simulink model "rfsoc4x2_ospfb_128"  (R2021a)
settings: Solver=VariableStepAuto  StartTime=0.0  StopTime=2048  RelTol=1e-3
undefined symbols (not defined in the file): pfb_coeff_gen_calc
libraries: xbsIndex_r4 x37092, casper_library_delays x737, casper_library_misc x68, xps_library x1
(part 232 of 339)

== system rfsoc4x2_ospfb_128/fft_wideband_real1/fft_direct/butterfly1_1/bus_convert/conv11 ==
  din : Inport
  all_0s : xbsIndex_r4/Logical  logical_function=NAND  inputs=3  en=off  latency=2  precision=Full  arith_type=Unsigned  n_bits=16  bin_pt=0  align_bp=on  dbl_ovrd=off  block_type=logical
  all_1s : xbsIndex_r4/Logical  logical_function=NAND  inputs=3  en=off  latency=2  precision=Full  arith_type=Unsigned  n_bits=16  bin_pt=0  align_bp=on  dbl_ovrd=off  block_type=logical
  and : xbsIndex_r4/Logical  logical_function=AND  inputs=2  en=off  latency=1  precision=Full  arith_type=Unsigned  n_bits=16  bin_pt=0  align_bp=on  dbl_ovrd=off  block_type=logical
  convert : xbsIndex_r4/Convert  gui_display_data_type=Fixed-point  arith_type="Signed  (2's comp)"  n_bits=bit_width_o  bin_pt=binary_point_o  float_type=Single  exp_bits=8  fraction_bits=24  quantization="Round  (unbiased: +/- Inf)"  overflow=Wrap  en=off  latency=csp_latency  pipeline=on  dbl_ovrd=off  block_type=convert
  invert1 : xbsIndex_r4/Inverter  en=off  latency=0  dbl_ovrd=off  block_type=inv
  invert2 : xbsIndex_r4/Inverter  en=off  latency=0  dbl_ovrd=off  block_type=inv
  invert3 : xbsIndex_r4/Inverter  en=off  latency=0  dbl_ovrd=off  block_type=inv
  slice1 : xbsIndex_r4/Slice  nbits=1  boolean_output=on  mode=Upper Bit Location + Width  bit1=0  base1=MSB of Input  bit0=0  base0=LSB of Input  dbl_ovrd=off  block_type=slice
  slice2 : xbsIndex_r4/Slice  nbits=1  boolean_output=on  mode=Upper Bit Location + Width  bit1=-1  base1=MSB of Input  bit0=0  base0=LSB of Input  dbl_ovrd=off  block_type=slice
  slice3 : xbsIndex_r4/Slice  nbits=1  boolean_output=on  mode=Upper Bit Location + Width  bit1=-2  base1=MSB of Input  bit0=0  base0=LSB of Input  dbl_ovrd=off  block_type=slice
  dout : Outport
  of : Outport  Port=2
  wires:
  and/1 -> of/1
  all_1s/1 -> and/2
  all_0s/1 -> and/1
  invert3/1 -> all_0s/3
  slice3/1 -> invert3/1, all_1s/3
  invert2/1 -> all_0s/2
  slice2/1 -> invert2/1, all_1s/2
  invert1/1 -> all_0s/1
  slice1/1 -> invert1/1, all_1s/1
  convert/1 -> dout/1
  din/1 -> slice3/1, slice2/1, slice1/1, convert/1

== system rfsoc4x2_ospfb_128/fft_wideband_real1/fft_direct/butterfly1_1/bus_convert/conv12 ==
  din : Inport
  all_0s : xbsIndex_r4/Logical  logical_function=NAND  inputs=3  en=off  latency=2  precision=Full  arith_type=Unsigned  n_bits=16  bin_pt=0  align_bp=on  dbl_ovrd=off  block_type=logical
  all_1s : xbsIndex_r4/Logical  logical_function=NAND  inputs=3  en=off  latency=2  precision=Full  arith_type=Unsigned  n_bits=16  bin_pt=0  align_bp=on  dbl_ovrd=off  block_type=logical
  and : xbsIndex_r4/Logical  logical_function=AND  inputs=2  en=off  latency=1  precision=Full  arith_type=Unsigned  n_bits=16  bin_pt=0  align_bp=on  dbl_ovrd=off  block_type=logical
  convert : xbsIndex_r4/Convert  gui_display_data_type=Fixed-point  arith_type="Signed  (2's comp)"  n_bits=bit_width_o  bin_pt=binary_point_o  float_type=Single  exp_bits=8  fraction_bits=24  quantization="Round  (unbiased: +/- Inf)"  overflow=Wrap  en=off  latency=csp_latency  pipeline=on  dbl_ovrd=off  block_type=convert
  invert1 : xbsIndex_r4/Inverter  en=off  latency=0  dbl_ovrd=off  block_type=inv
  invert2 : xbsIndex_r4/Inverter  en=off  latency=0  dbl_ovrd=off  block_type=inv
  invert3 : xbsIndex_r4/Inverter  en=off  latency=0  dbl_ovrd=off  block_type=inv
  slice1 : xbsIndex_r4/Slice  nbits=1  boolean_output=on  mode=Upper Bit Location + Width  bit1=0  base1=MSB of Input  bit0=0  base0=LSB of Input  dbl_ovrd=off  block_type=slice
  slice2 : xbsIndex_r4/Slice  nbits=1  boolean_output=on  mode=Upper Bit Location + Width  bit1=-1  base1=MSB of Input  bit0=0  base0=LSB of Input  dbl_ovrd=off  block_type=slice
  slice3 : xbsIndex_r4/Slice  nbits=1  boolean_output=on  mode=Upper Bit Location + Width  bit1=-2  base1=MSB of Input  bit0=0  base0=LSB of Input  dbl_ovrd=off  block_type=slice
  dout : Outport
  of : Outport  Port=2
  wires:
  and/1 -> of/1
  all_1s/1 -> and/2
  all_0s/1 -> and/1
  invert3/1 -> all_0s/3
  slice3/1 -> invert3/1, all_1s/3
  invert2/1 -> all_0s/2
  slice2/1 -> invert2/1, all_1s/2
  invert1/1 -> all_0s/1
  slice1/1 -> invert1/1, all_1s/1
  convert/1 -> dout/1
  din/1 -> slice3/1, slice2/1, slice1/1, convert/1

== system rfsoc4x2_ospfb_128/fft_wideband_real1/fft_direct/butterfly1_1/bus_convert/conv13 ==
  din : Inport
  all_0s : xbsIndex_r4/Logical  logical_function=NAND  inputs=3  en=off  latency=2  precision=Full  arith_type=Unsigned  n_bits=16  bin_pt=0  align_bp=on  dbl_ovrd=off  block_type=logical
  all_1s : xbsIndex_r4/Logical  logical_function=NAND  inputs=3  en=off  latency=2  precision=Full  arith_type=Unsigned  n_bits=16  bin_pt=0  align_bp=on  dbl_ovrd=off  block_type=logical
  and : xbsIndex_r4/Logical  logical_function=AND  inputs=2  en=off  latency=1  precision=Full  arith_type=Unsigned  n_bits=16  bin_pt=0  align_bp=on  dbl_ovrd=off  block_type=logical
  convert : xbsIndex_r4/Convert  gui_display_data_type=Fixed-point  arith_type="Signed  (2's comp)"  n_bits=bit_width_o  bin_pt=binary_point_o  float_type=Single  exp_bits=8  fraction_bits=24  quantization="Round  (unbiased: +/- Inf)"  overflow=Wrap  en=off  latency=csp_latency  pipeline=on  dbl_ovrd=off  block_type=convert
  invert1 : xbsIndex_r4/Inverter  en=off  latency=0  dbl_ovrd=off  block_type=inv
  invert2 : xbsIndex_r4/Inverter  en=off  latency=0  dbl_ovrd=off  block_type=inv
  invert3 : xbsIndex_r4/Inverter  en=off  latency=0  dbl_ovrd=off  block_type=inv
  slice1 : xbsIndex_r4/Slice  nbits=1  boolean_output=on  mode=Upper Bit Location + Width  bit1=0  base1=MSB of Input  bit0=0  base0=LSB of Input  dbl_ovrd=off  block_type=slice
  slice2 : xbsIndex_r4/Slice  nbits=1  boolean_output=on  mode=Upper Bit Location + Width  bit1=-1  base1=MSB of Input  bit0=0  base0=LSB of Input  dbl_ovrd=off  block_type=slice
  slice3 : xbsIndex_r4/Slice  nbits=1  boolean_output=on  mode=Upper Bit Location + Width  bit1=-2  base1=MSB of Input  bit0=0  base0=LSB of Input  dbl_ovrd=off  block_type=slice
  dout : Outport
  of : Outport  Port=2
  wires:
  and/1 -> of/1
  all_1s/1 -> and/2
  all_0s/1 -> and/1
  invert3/1 -> all_0s/3
  slice3/1 -> invert3/1, all_1s/3
  invert2/1 -> all_0s/2
  slice2/1 -> invert2/1, all_1s/2
  invert1/1 -> all_0s/1
  slice1/1 -> invert1/1, all_1s/1
  convert/1 -> dout/1
  din/1 -> slice3/1, slice2/1, slice1/1, convert/1

== system rfsoc4x2_ospfb_128/fft_wideband_real1/fft_direct/butterfly1_1/bus_convert/conv14 ==
  din : Inport
  all_0s : xbsIndex_r4/Logical  logical_function=NAND  inputs=3  en=off  latency=2  precision=Full  arith_type=Unsigned  n_bits=16  bin_pt=0  align_bp=on  dbl_ovrd=off  block_type=logical
  all_1s : xbsIndex_r4/Logical  logical_function=NAND  inputs=3  en=off  latency=2  precision=Full  arith_type=Unsigned  n_bits=16  bin_pt=0  align_bp=on  dbl_ovrd=off  block_type=logical
  and : xbsIndex_r4/Logical  logical_function=AND  inputs=2  en=off  latency=1  precision=Full  arith_type=Unsigned  n_bits=16  bin_pt=0  align_bp=on  dbl_ovrd=off  block_type=logical
  convert : xbsIndex_r4/Convert  gui_display_data_type=Fixed-point  arith_type="Signed  (2's comp)"  n_bits=bit_width_o  bin_pt=binary_point_o  float_type=Single  exp_bits=8  fraction_bits=24  quantization="Round  (unbiased: +/- Inf)"  overflow=Wrap  en=off  latency=csp_latency  pipeline=on  dbl_ovrd=off  block_type=convert
  invert1 : xbsIndex_r4/Inverter  en=off  latency=0  dbl_ovrd=off  block_type=inv
  invert2 : xbsIndex_r4/Inverter  en=off  latency=0  dbl_ovrd=off  block_type=inv
  invert3 : xbsIndex_r4/Inverter  en=off  latency=0  dbl_ovrd=off  block_type=inv
  slice1 : xbsIndex_r4/Slice  nbits=1  boolean_output=on  mode=Upper Bit Location + Width  bit1=0  base1=MSB of Input  bit0=0  base0=LSB of Input  dbl_ovrd=off  block_type=slice
  slice2 : xbsIndex_r4/Slice  nbits=1  boolean_output=on  mode=Upper Bit Location + Width  bit1=-1  base1=MSB of Input  bit0=0  base0=LSB of Input  dbl_ovrd=off  block_type=slice
  slice3 : xbsIndex_r4/Slice  nbits=1  boolean_output=on  mode=Upper Bit Location + Width  bit1=-2  base1=MSB of Input  bit0=0  base0=LSB of Input  dbl_ovrd=off  block_type=slice
  dout : Outport
  of : Outport  Port=2
  wires:
  and/1 -> of/1
  all_1s/1 -> and/2
  all_0s/1 -> and/1
  invert3/1 -> all_0s/3
  slice3/1 -> invert3/1, all_1s/3
  invert2/1 -> all_0s/2
  slice2/1 -> invert2/1, all_1s/2
  invert1/1 -> all_0s/1
  slice1/1 -> invert1/1, all_1s/1
  convert/1 -> dout/1
  din/1 -> slice3/1, slice2/1, slice1/1, convert/1

== system rfsoc4x2_ospfb_128/fft_wideband_real1/fft_direct/butterfly1_1/bus_convert/conv15 ==
  din : Inport
  all_0s : xbsIndex_r4/Logical  logical_function=NAND  inputs=3  en=off  latency=2  precision=Full  arith_type=Unsigned  n_bits=16  bin_pt=0  align_bp=on  dbl_ovrd=off  block_type=logical
  all_1s : xbsIndex_r4/Logical  logical_function=NAND  inputs=3  en=off  latency=2  precision=Full  arith_type=Unsigned  n_bits=16  bin_pt=0  align_bp=on  dbl_ovrd=off  block_type=logical
  and : xbsIndex_r4/Logical  logical_function=AND  inputs=2  en=off  latency=1  precision=Full  arith_type=Unsigned  n_bits=16  bin_pt=0  align_bp=on  dbl_ovrd=off  block_type=logical
  convert : xbsIndex_r4/Convert  gui_display_data_type=Fixed-point  arith_type="Signed  (2's comp)"  n_bits=bit_width_o  bin_pt=binary_point_o  float_type=Single  exp_bits=8  fraction_bits=24  quantization="Round  (unbiased: +/- Inf)"  overflow=Wrap  en=off  latency=csp_latency  pipeline=on  dbl_ovrd=off  block_type=convert
  invert1 : xbsIndex_r4/Inverter  en=off  latency=0  dbl_ovrd=off  block_type=inv
  invert2 : xbsIndex_r4/Inverter  en=off  latency=0  dbl_ovrd=off  block_type=inv
  invert3 : xbsIndex_r4/Inverter  en=off  latency=0  dbl_ovrd=off  block_type=inv
  slice1 : xbsIndex_r4/Slice  nbits=1  boolean_output=on  mode=Upper Bit Location + Width  bit1=0  base1=MSB of Input  bit0=0  base0=LSB of Input  dbl_ovrd=off  block_type=slice
  slice2 : xbsIndex_r4/Slice  nbits=1  boolean_output=on  mode=Upper Bit Location + Width  bit1=-1  base1=MSB of Input  bit0=0  base0=LSB of Input  dbl_ovrd=off  block_type=slice
  slice3 : xbsIndex_r4/Slice  nbits=1  boolean_output=on  mode=Upper Bit Location + Width  bit1=-2  base1=MSB of Input  bit0=0  base0=LSB of Input  dbl_ovrd=off  block_type=slice
  dout : Outport
  of : Outport  Port=2
  wires:
  and/1 -> of/1
  all_1s/1 -> and/2
  all_0s/1 -> and/1
  invert3/1 -> all_0s/3
  slice3/1 -> invert3/1, all_1s/3
  invert2/1 -> all_0s/2
  slice2/1 -> invert2/1, all_1s/2
  invert1/1 -> all_0s/1
  slice1/1 -> invert1/1, all_1s/1
  convert/1 -> dout/1
  din/1 -> slice3/1, slice2/1, slice1/1, convert/1

== system rfsoc4x2_ospfb_128/fft_wideband_real1/fft_direct/butterfly1_1/bus_convert/conv16 ==
  din : Inport
  all_0s : xbsIndex_r4/Logical  logical_function=NAND  inputs=3  en=off  latency=2  precision=Full  arith_type=Unsigned  n_bits=16  bin_pt=0  align_bp=on  dbl_ovrd=off  block_type=logical
  all_1s : xbsIndex_r4/Logical  logical_function=NAND  inputs=3  en=off  latency=2  precision=Full  arith_type=Unsigned  n_bits=16  bin_pt=0  align_bp=on  dbl_ovrd=off  block_type=logical
  and : xbsIndex_r4/Logical  logical_function=AND  inputs=2  en=off  latency=1  precision=Full  arith_type=Unsigned  n_bits=16  bin_pt=0  align_bp=on  dbl_ovrd=off  block_type=logical
  convert : xbsIndex_r4/Convert  gui_display_data_type=Fixed-point  arith_type="Signed  (2's comp)"  n_bits=bit_width_o  bin_pt=binary_point_o  float_type=Single  exp_bits=8  fraction_bits=24  quantization="Round  (unbiased: +/- Inf)"  overflow=Wrap  en=off  latency=csp_latency  pipeline=on  dbl_ovrd=off  block_type=convert
  invert1 : xbsIndex_r4/Inverter  en=off  latency=0  dbl_ovrd=off  block_type=inv
  invert2 : xbsIndex_r4/Inverter  en=off  latency=0  dbl_ovrd=off  block_type=inv
  invert3 : xbsIndex_r4/Inverter  en=off  latency=0  dbl_ovrd=off  block_type=inv
  slice1 : xbsIndex_r4/Slice  nbits=1  boolean_output=on  mode=Upper Bit Location + Width  bit1=0  base1=MSB of Input  bit0=0  base0=LSB of Input  dbl_ovrd=off  block_type=slice
  slice2 : xbsIndex_r4/Slice  nbits=1  boolean_output=on  mode=Upper Bit Location + Width  bit1=-1  base1=MSB of Input  bit0=0  base0=LSB of Input  dbl_ovrd=off  block_type=slice
  slice3 : xbsIndex_r4/Slice  nbits=1  boolean_output=on  mode=Upper Bit Location + Width  bit1=-2  base1=MSB of Input  bit0=0  base0=LSB of Input  dbl_ovrd=off  block_type=slice
  dout : Outport
  of : Outport  Port=2
  wires:
  and/1 -> of/1
  all_1s/1 -> and/2
  all_0s/1 -> and/1
  invert3/1 -> all_0s/3
  slice3/1 -> invert3/1, all_1s/3
  invert2/1 -> all_0s/2
  slice2/1 -> invert2/1, all_1s/2
  invert1/1 -> all_0s/1
  slice1/1 -> invert1/1, all_1s/1
  convert/1 -> dout/1
  din/1 -> slice3/1, slice2/1, slice1/1, convert/1

== system rfsoc4x2_ospfb_128/fft_wideband_real1/fft_direct/butterfly1_1/bus_convert/conv2 ==
  din : Inport
  all_0s : xbsIndex_r4/Logical  logical_function=NAND  inputs=3  en=off  latency=2  precision=Full  arith_type=Unsigned  n_bits=16  bin_pt=0  align_bp=on  dbl_ovrd=off  block_type=logical
  all_1s : xbsIndex_r4/Logical  logical_function=NAND  inputs=3  en=off  latency=2  precision=Full  arith_type=Unsigned  n_bits=16  bin_pt=0  align_bp=on  dbl_ovrd=off  block_type=logical
  and : xbsIndex_r4/Logical  logical_function=AND  inputs=2  en=off  latency=1  precision=Full  arith_type=Unsigned  n_bits=16  bin_pt=0  align_bp=on  dbl_ovrd=off  block_type=logical
  convert : xbsIndex_r4/Convert  gui_display_data_type=Fixed-point  arith_type="Signed  (2's comp)"  n_bits=bit_width_o  bin_pt=binary_point_o  float_type=Single  exp_bits=8  fraction_bits=24  quantization="Round  (unbiased: +/- Inf)"  overflow=Wrap  en=off  latency=csp_latency  pipeline=on  dbl_ovrd=off  block_type=convert
  invert1 : xbsIndex_r4/Inverter  en=off  latency=0  dbl_ovrd=off  block_type=inv
  invert2 : xbsIndex_r4/Inverter  en=off  latency=0  dbl_ovrd=off  block_type=inv
  invert3 : xbsIndex_r4/Inverter  en=off  latency=0  dbl_ovrd=off  block_type=inv
  slice1 : xbsIndex_r4/Slice  nbits=1  boolean_output=on  mode=Upper Bit Location + Width  bit1=0  base1=MSB of Input  bit0=0  base0=LSB of Input  dbl_ovrd=off  block_type=slice
  slice2 : xbsIndex_r4/Slice  nbits=1  boolean_output=on  mode=Upper Bit Location + Width  bit1=-1  base1=MSB of Input  bit0=0  base0=LSB of Input  dbl_ovrd=off  block_type=slice
  slice3 : xbsIndex_r4/Slice  nbits=1  boolean_output=on  mode=Upper Bit Location + Width  bit1=-2  base1=MSB of Input  bit0=0  base0=LSB of Input  dbl_ovrd=off  block_type=slice
  dout : Outport
  of : Outport  Port=2
  wires:
  and/1 -> of/1
  all_1s/1 -> and/2
  all_0s/1 -> and/1
  invert3/1 -> all_0s/3
  slice3/1 -> invert3/1, all_1s/3
  invert2/1 -> all_0s/2
  slice2/1 -> invert2/1, all_1s/2
  invert1/1 -> all_0s/1
  slice1/1 -> invert1/1, all_1s/1
  convert/1 -> dout/1
  din/1 -> slice3/1, slice2/1, slice1/1, convert/1

== system rfsoc4x2_ospfb_128/fft_wideband_real1/fft_direct/butterfly1_1/bus_convert/conv3 ==
  din : Inport
  all_0s : xbsIndex_r4/Logical  logical_function=NAND  inputs=3  en=off  latency=2  precision=Full  arith_type=Unsigned  n_bits=16  bin_pt=0  align_bp=on  dbl_ovrd=off  block_type=logical
  all_1s : xbsIndex_r4/Logical  logical_function=NAND  inputs=3  en=off  latency=2  precision=Full  arith_type=Unsigned  n_bits=16  bin_pt=0  align_bp=on  dbl_ovrd=off  block_type=logical
  and : xbsIndex_r4/Logical  logical_function=AND  inputs=2  en=off  latency=1  precision=Full  arith_type=Unsigned  n_bits=16  bin_pt=0  align_bp=on  dbl_ovrd=off  block_type=logical
  convert : xbsIndex_r4/Convert  gui_display_data_type=Fixed-point  arith_type="Signed  (2's comp)"  n_bits=bit_width_o  bin_pt=binary_point_o  float_type=Single  exp_bits=8  fraction_bits=24  quantization="Round  (unbiased: +/- Inf)"  overflow=Wrap  en=off  latency=csp_latency  pipeline=on  dbl_ovrd=off  block_type=convert
  invert1 : xbsIndex_r4/Inverter  en=off  latency=0  dbl_ovrd=off  block_type=inv
  invert2 : xbsIndex_r4/Inverter  en=off  latency=0  dbl_ovrd=off  block_type=inv
  invert3 : xbsIndex_r4/Inverter  en=off  latency=0  dbl_ovrd=off  block_type=inv
  slice1 : xbsIndex_r4/Slice  nbits=1  boolean_output=on  mode=Upper Bit Location + Width  bit1=0  base1=MSB of Input  bit0=0  base0=LSB of Input  dbl_ovrd=off  block_type=slice
  slice2 : xbsIndex_r4/Slice  nbits=1  boolean_output=on  mode=Upper Bit Location + Width  bit1=-1  base1=MSB of Input  bit0=0  base0=LSB of Input  dbl_ovrd=off  block_type=slice
  slice3 : xbsIndex_r4/Slice  nbits=1  boolean_output=on  mode=Upper Bit Location + Width  bit1=-2  base1=MSB of Input  bit0=0  base0=LSB of Input  dbl_ovrd=off  block_type=slice
  dout : Outport
  of : Outport  Port=2
  wires:
  and/1 -> of/1
  all_1s/1 -> and/2
  all_0s/1 -> and/1
  invert3/1 -> all_0s/3
  slice3/1 -> invert3/1, all_1s/3
  invert2/1 -> all_0s/2
  slice2/1 -> invert2/1, all_1s/2
  invert1/1 -> all_0s/1
  slice1/1 -> invert1/1, all_1s/1
  convert/1 -> dout/1
  din/1 -> slice3/1, slice2/1, slice1/1, convert/1

== system rfsoc4x2_ospfb_128/fft_wideband_real1/fft_direct/butterfly1_1/bus_convert/conv4 ==
  din : Inport
  all_0s : xbsIndex_r4/Logical  logical_function=NAND  inputs=3  en=off  latency=2  precision=Full  arith_type=Unsigned  n_bits=16  bin_pt=0  align_bp=on  dbl_ovrd=off  block_type=logical
  all_1s : xbsIndex_r4/Logical  logical_function=NAND  inputs=3  en=off  latency=2  precision=Full  arith_type=Unsigned  n_bits=16  bin_pt=0  align_bp=on  dbl_ovrd=off  block_type=logical
  and : xbsIndex_r4/Logical  logical_function=AND  inputs=2  en=off  latency=1  precision=Full  arith_type=Unsigned  n_bits=16  bin_pt=0  align_bp=on  dbl_ovrd=off  block_type=logical
  convert : xbsIndex_r4/Convert  gui_display_data_type=Fixed-point  arith_type="Signed  (2's comp)"  n_bits=bit_width_o  bin_pt=binary_point_o  float_type=Single  exp_bits=8  fraction_bits=24  quantization="Round  (unbiased: +/- Inf)"  overflow=Wrap  en=off  latency=csp_latency  pipeline=on  dbl_ovrd=off  block_type=convert
  invert1 : xbsIndex_r4/Inverter  en=off  latency=0  dbl_ovrd=off  block_type=inv
  invert2 : xbsIndex_r4/Inverter  en=off  latency=0  dbl_ovrd=off  block_type=inv
  invert3 : xbsIndex_r4/Inverter  en=off  latency=0  dbl_ovrd=off  block_type=inv
  slice1 : xbsIndex_r4/Slice  nbits=1  boolean_output=on  mode=Upper Bit Location + Width  bit1=0  base1=MSB of Input  bit0=0  base0=LSB of Input  dbl_ovrd=off  block_type=slice
  slice2 : xbsIndex_r4/Slice  nbits=1  boolean_output=on  mode=Upper Bit Location + Width  bit1=-1  base1=MSB of Input  bit0=0  base0=LSB of Input  dbl_ovrd=off  block_type=slice
  slice3 : xbsIndex_r4/Slice  nbits=1  boolean_output=on  mode=Upper Bit Location + Width  bit1=-2  base1=MSB of Input  bit0=0  base0=LSB of Input  dbl_ovrd=off  block_type=slice
  dout : Outport
  of : Outport  Port=2
  wires:
  and/1 -> of/1
  all_1s/1 -> and/2
  all_0s/1 -> and/1
  invert3/1 -> all_0s/3
  slice3/1 -> invert3/1, all_1s/3
  invert2/1 -> all_0s/2
  slice2/1 -> invert2/1, all_1s/2
  invert1/1 -> all_0s/1
  slice1/1 -> invert1/1, all_1s/1
  convert/1 -> dout/1
  din/1 -> slice3/1, slice2/1, slice1/1, convert/1

== system rfsoc4x2_ospfb_128/fft_wideband_real1/fft_direct/butterfly1_1/bus_convert/conv5 ==
  din : Inport
  all_0s : xbsIndex_r4/Logical  logical_function=NAND  inputs=3  en=off  latency=2  precision=Full  arith_type=Unsigned  n_bits=16  bin_pt=0  align_bp=on  dbl_ovrd=off  block_type=logical
  all_1s : xbsIndex_r4/Logical  logical_function=NAND  inputs=3  en=off  latency=2  precision=Full  arith_type=Unsigned  n_bits=16  bin_pt=0  align_bp=on  dbl_ovrd=off  block_type=logical
  and : xbsIndex_r4/Logical  logical_function=AND  inputs=2  en=off  latency=1  precision=Full  arith_type=Unsigned  n_bits=16  bin_pt=0  align_bp=on  dbl_ovrd=off  block_type=logical
  convert : xbsIndex_r4/Convert  gui_display_data_type=Fixed-point  arith_type="Signed  (2's comp)"  n_bits=bit_width_o  bin_pt=binary_point_o  float_type=Single  exp_bits=8  fraction_bits=24  quantization="Round  (unbiased: +/- Inf)"  overflow=Wrap  en=off  latency=csp_latency  pipeline=on  dbl_ovrd=off  block_type=convert
  invert1 : xbsIndex_r4/Inverter  en=off  latency=0  dbl_ovrd=off  block_type=inv
  invert2 : xbsIndex_r4/Inverter  en=off  latency=0  dbl_ovrd=off  block_type=inv
  invert3 : xbsIndex_r4/Inverter  en=off  latency=0  dbl_ovrd=off  block_type=inv
  slice1 : xbsIndex_r4/Slice  nbits=1  boolean_output=on  mode=Upper Bit Location + Width  bit1=0  base1=MSB of Input  bit0=0  base0=LSB of Input  dbl_ovrd=off  block_type=slice
  slice2 : xbsIndex_r4/Slice  nbits=1  boolean_output=on  mode=Upper Bit Location + Width  bit1=-1  base1=MSB of Input  bit0=0  base0=LSB of Input  dbl_ovrd=off  block_type=slice
  slice3 : xbsIndex_r4/Slice  nbits=1  boolean_output=on  mode=Upper Bit Location + Width  bit1=-2  base1=MSB of Input  bit0=0  base0=LSB of Input  dbl_ovrd=off  block_type=slice
  dout : Outport
  of : Outport  Port=2
  wires:
  and/1 -> of/1
  all_1s/1 -> and/2
  all_0s/1 -> and/1
  invert3/1 -> all_0s/3
  slice3/1 -> invert3/1, all_1s/3
  invert2/1 -> all_0s/2
  slice2/1 -> invert2/1, all_1s/2
  invert1/1 -> all_0s/1
  slice1/1 -> invert1/1, all_1s/1
  convert/1 -> dout/1
  din/1 -> slice3/1, slice2/1, slice1/1, convert/1

== system rfsoc4x2_ospfb_128/fft_wideband_real1/fft_direct/butterfly1_1/bus_convert/conv6 ==
  din : Inport
  all_0s : xbsIndex_r4/Logical  logical_function=NAND  inputs=3  en=off  latency=2  precision=Full  arith_type=Unsigned  n_bits=16  bin_pt=0  align_bp=on  dbl_ovrd=off  block_type=logical
  all_1s : xbsIndex_r4/Logical  logical_function=NAND  inputs=3  en=off  latency=2  precision=Full  arith_type=Unsigned  n_bits=16  bin_pt=0  align_bp=on  dbl_ovrd=off  block_type=logical
  and : xbsIndex_r4/Logical  logical_function=AND  inputs=2  en=off  latency=1  precision=Full  arith_type=Unsigned  n_bits=16  bin_pt=0  align_bp=on  dbl_ovrd=off  block_type=logical
  convert : xbsIndex_r4/Convert  gui_display_data_type=Fixed-point  arith_type="Signed  (2's comp)"  n_bits=bit_width_o  bin_pt=binary_point_o  float_type=Single  exp_bits=8  fraction_bits=24  quantization="Round  (unbiased: +/- Inf)"  overflow=Wrap  en=off  latency=csp_latency  pipeline=on  dbl_ovrd=off  block_type=convert
  invert1 : xbsIndex_r4/Inverter  en=off  latency=0  dbl_ovrd=off  block_type=inv
  invert2 : xbsIndex_r4/Inverter  en=off  latency=0  dbl_ovrd=off  block_type=inv
  invert3 : xbsIndex_r4/Inverter  en=off  latency=0  dbl_ovrd=off  block_type=inv
  slice1 : xbsIndex_r4/Slice  nbits=1  boolean_output=on  mode=Upper Bit Location + Width  bit1=0  base1=MSB of Input  bit0=0  base0=LSB of Input  dbl_ovrd=off  block_type=slice
  slice2 : xbsIndex_r4/Slice  nbits=1  boolean_output=on  mode=Upper Bit Location + Width  bit1=-1  base1=MSB of Input  bit0=0  base0=LSB of Input  dbl_ovrd=off  block_type=slice
  slice3 : xbsIndex_r4/Slice  nbits=1  boolean_output=on  mode=Upper Bit Location + Width  bit1=-2  base1=MSB of Input  bit0=0  base0=LSB of Input  dbl_ovrd=off  block_type=slice
  dout : Outport
  of : Outport  Port=2
  wires:
  and/1 -> of/1
  all_1s/1 -> and/2
  all_0s/1 -> and/1
  invert3/1 -> all_0s/3
  slice3/1 -> invert3/1, all_1s/3
  invert2/1 -> all_0s/2
  slice2/1 -> invert2/1, all_1s/2
  invert1/1 -> all_0s/1
  slice1/1 -> invert1/1, all_1s/1
  convert/1 -> dout/1
  din/1 -> slice3/1, slice2/1, slice1/1, convert/1

== system rfsoc4x2_ospfb_128/fft_wideband_real1/fft_direct/butterfly1_1/bus_convert/conv7 ==
  din : Inport
  all_0s : xbsIndex_r4/Logical  logical_function=NAND  inputs=3  en=off  latency=2  precision=Full  arith_type=Unsigned  n_bits=16  bin_pt=0  align_bp=on  dbl_ovrd=off  block_type=logical
  all_1s : xbsIndex_r4/Logical  logical_function=NAND  inputs=3  en=off  latency=2  precision=Full  arith_type=Unsigned  n_bits=16  bin_pt=0  align_bp=on  dbl_ovrd=off  block_type=logical
  and : xbsIndex_r4/Logical  logical_function=AND  inputs=2  en=off  latency=1  precision=Full  arith_type=Unsigned  n_bits=16  bin_pt=0  align_bp=on  dbl_ovrd=off  block_type=logical
  convert : xbsIndex_r4/Convert  gui_display_data_type=Fixed-point  arith_type="Signed  (2's comp)"  n_bits=bit_width_o  bin_pt=binary_point_o  float_type=Single  exp_bits=8  fraction_bits=24  quantization="Round  (unbiased: +/- Inf)"  overflow=Wrap  en=off  latency=csp_latency  pipeline=on  dbl_ovrd=off  block_type=convert
  invert1 : xbsIndex_r4/Inverter  en=off  latency=0  dbl_ovrd=off  block_type=inv
  invert2 : xbsIndex_r4/Inverter  en=off  latency=0  dbl_ovrd=off  block_type=inv
  invert3 : xbsIndex_r4/Inverter  en=off  latency=0  dbl_ovrd=off  block_type=inv
  slice1 : xbsIndex_r4/Slice  nbits=1  boolean_output=on  mode=Upper Bit Location + Width  bit1=0  base1=MSB of Input  bit0=0  base0=LSB of Input  dbl_ovrd=off  block_type=slice
  slice2 : xbsIndex_r4/Slice  nbits=1  boolean_output=on  mode=Upper Bit Location + Width  bit1=-1  base1=MSB of Input  bit0=0  base0=LSB of Input  dbl_ovrd=off  block_type=slice
  slice3 : xbsIndex_r4/Slice  nbits=1  boolean_output=on  mode=Upper Bit Location + Width  bit1=-2  base1=MSB of Input  bit0=0  base0=LSB of Input  dbl_ovrd=off  block_type=slice
  dout : Outport
  of : Outport  Port=2
  wires:
  and/1 -> of/1
  all_1s/1 -> and/2
  all_0s/1 -> and/1
  invert3/1 -> all_0s/3
  slice3/1 -> invert3/1, all_1s/3
  invert2/1 -> all_0s/2
  slice2/1 -> invert2/1, all_1s/2
  invert1/1 -> all_0s/1
  slice1/1 -> invert1/1, all_1s/1
  convert/1 -> dout/1
  din/1 -> slice3/1, slice2/1, slice1/1, convert/1

== system rfsoc4x2_ospfb_128/fft_wideband_real1/fft_direct/butterfly1_1/bus_convert/conv8 ==
  din : Inport
  all_0s : xbsIndex_r4/Logical  logical_function=NAND  inputs=3  en=off  latency=2  precision=Full  arith_type=Unsigned  n_bits=16  bin_pt=0  align_bp=on  dbl_ovrd=off  block_type=logical
  all_1s : xbsIndex_r4/Logical  logical_function=NAND  inputs=3  en=off  latency=2  precision=Full  arith_type=Unsigned  n_bits=16  bin_pt=0  align_bp=on  dbl_ovrd=off  block_type=logical
  and : xbsIndex_r4/Logical  logical_function=AND  inputs=2  en=off  latency=1  precision=Full  arith_type=Unsigned  n_bits=16  bin_pt=0  align_bp=on  dbl_ovrd=off  block_type=logical
  convert : xbsIndex_r4/Convert  gui_display_data_type=Fixed-point  arith_type="Signed  (2's comp)"  n_bits=bit_width_o  bin_pt=binary_point_o  float_type=Single  exp_bits=8  fraction_bits=24  quantization="Round  (unbiased: +/- Inf)"  overflow=Wrap  en=off  latency=csp_latency  pipeline=on  dbl_ovrd=off  block_type=convert
  invert1 : xbsIndex_r4/Inverter  en=off  latency=0  dbl_ovrd=off  block_type=inv
  invert2 : xbsIndex_r4/Inverter  en=off  latency=0  dbl_ovrd=off  block_type=inv
  invert3 : xbsIndex_r4/Inverter  en=off  latency=0  dbl_ovrd=off  block_type=inv
  slice1 : xbsIndex_r4/Slice  nbits=1  boolean_output=on  mode=Upper Bit Location + Width  bit1=0  base1=MSB of Input  bit0=0  base0=LSB of Input  dbl_ovrd=off  block_type=slice
  slice2 : xbsIndex_r4/Slice  nbits=1  boolean_output=on  mode=Upper Bit Location + Width  bit1=-1  base1=MSB of Input  bit0=0  base0=LSB of Input  dbl_ovrd=off  block_type=slice
  slice3 : xbsIndex_r4/Slice  nbits=1  boolean_output=on  mode=Upper Bit Location + Width  bit1=-2  base1=MSB of Input  bit0=0  base0=LSB of Input  dbl_ovrd=off  block_type=slice
  dout : Outport
  of : Outport  Port=2
  wires:
  and/1 -> of/1
  all_1s/1 -> and/2
  all_0s/1 -> and/1
  invert3/1 -> all_0s/3
  slice3/1 -> invert3/1, all_1s/3
  invert2/1 -> all_0s/2
  slice2/1 -> invert2/1, all_1s/2
  invert1/1 -> all_0s/1
  slice1/1 -> invert1/1, all_1s/1
  convert/1 -> dout/1
  din/1 -> slice3/1, slice2/1, slice1/1, convert/1

== system rfsoc4x2_ospfb_128/fft_wideband_real1/fft_direct/butterfly1_1/bus_convert/conv9 ==
  din : Inport
  all_0s : xbsIndex_r4/Logical  logical_function=NAND  inputs=3  en=off  latency=2  precision=Full  arith_type=Unsigned  n_bits=16  bin_pt=0  align_bp=on  dbl_ovrd=off  block_type=logical
  all_1s : xbsIndex_r4/Logical  logical_function=NAND  inputs=3  en=off  latency=2  precision=Full  arith_type=Unsigned  n_bits=16  bin_pt=0  align_bp=on  dbl_ovrd=off  block_type=logical
  and : xbsIndex_r4/Logical  logical_function=AND  inputs=2  en=off  latency=1  precision=Full  arith_type=Unsigned  n_bits=16  bin_pt=0  align_bp=on  dbl_ovrd=off  block_type=logical
  convert : xbsIndex_r4/Convert  gui_display_data_type=Fixed-point  arith_type="Signed  (2's comp)"  n_bits=bit_width_o  bin_pt=binary_point_o  float_type=Single  exp_bits=8  fraction_bits=24  quantization="Round  (unbiased: +/- Inf)"  overflow=Wrap  en=off  latency=csp_latency  pipeline=on  dbl_ovrd=off  block_type=convert
  invert1 : xbsIndex_r4/Inverter  en=off  latency=0  dbl_ovrd=off  block_type=inv
  invert2 : xbsIndex_r4/Inverter  en=off  latency=0  dbl_ovrd=off  block_type=inv
  invert3 : xbsIndex_r4/Inverter  en=off  latency=0  dbl_ovrd=off  block_type=inv
  slice1 : xbsIndex_r4/Slice  nbits=1  boolean_output=on  mode=Upper Bit Location + Width  bit1=0  base1=MSB of Input  bit0=0  base0=LSB of Input  dbl_ovrd=off  block_type=slice
  slice2 : xbsIndex_r4/Slice  nbits=1  boolean_output=on  mode=Upper Bit Location + Width  bit1=-1  base1=MSB of Input  bit0=0  base0=LSB of Input  dbl_ovrd=off  block_type=slice
  slice3 : xbsIndex_r4/Slice  nbits=1  boolean_output=on  mode=Upper Bit Location + Width  bit1=-2  base1=MSB of Input  bit0=0  base0=LSB of Input  dbl_ovrd=off  block_type=slice
  dout : Outport
  of : Outport  Port=2
  wires:
  and/1 -> of/1
  all_1s/1 -> and/2
  all_0s/1 -> and/1
  invert3/1 -> all_0s/3
  slice3/1 -> invert3/1, all_1s/3
  invert2/1 -> all_0s/2
  slice2/1 -> invert2/1, all_1s/2
  invert1/1 -> all_0s/1
  slice1/1 -> invert1/1, all_1s/1
  convert/1 -> dout/1
  din/1 -> slice3/1, slice2/1, slice1/1, convert/1

== system rfsoc4x2_ospfb_128/fft_wideband_real1/fft_direct/butterfly1_1/bus_convert/debus ==
  bus_in : Inport
  reinterpret{1..16} (16 alike) : xbsIndex_r4/Reinterpret  force_arith_type=on  arith_type="Signed  (2's comp)"  force_bin_pt=on  bin_pt=18  block_type=reinterpret
  slice1 : xbsIndex_r4/Slice  nbits=21  boolean_output=off  mode=Upper Bit Location + Width  bit1=-315  base1=MSB of Input  bit0=0  base0=LSB of Input  dbl_ovrd=off  block_type=slice
  slice10 : xbsIndex_r4/Slice  nbits=21  boolean_output=off  mode=Upper Bit Location + Width  bit1=-126  base1=MSB of Input  bit0=0  base0=LSB of Input  dbl_ovrd=off  block_type=slice
  slice11 : xbsIndex_r4/Slice  nbits=21  boolean_output=off  mode=Upper Bit Location + Width  bit1=-105  base1=MSB of Input  bit0=0  base0=LSB of Input  dbl_ovrd=off  block_type=slice
  slice12 : xbsIndex_r4/Slice  nbits=21  boolean_output=off  mode=Upper Bit Location + Width  bit1=-84  base1=MSB of Input  bit0=0  base0=LSB of Input  dbl_ovrd=off  block_type=slice
  slice13 : xbsIndex_r4/Slice  nbits=21  boolean_output=off  mode=Upper Bit Location + Width  bit1=-63  base1=MSB of Input  bit0=0  base0=LSB of Input  dbl_ovrd=off  block_type=slice
  slice14 : xbsIndex_r4/Slice  nbits=21  boolean_output=off  mode=Upper Bit Location + Width  bit1=-42  base1=MSB of Input  bit0=0  base0=LSB of Input  dbl_ovrd=off  block_type=slice
  slice15 : xbsIndex_r4/Slice  nbits=21  boolean_output=off  mode=Upper Bit Location + Width  bit1=-21  base1=MSB of Input  bit0=0  base0=LSB of Input  dbl_ovrd=off  block_type=slice
  slice16 : xbsIndex_r4/Slice  nbits=21  boolean_output=off  mode=Upper Bit Location + Width  bit1=0  base1=MSB of Input  bit0=0  base0=LSB of Input  dbl_ovrd=off  block_type=slice
  slice2 : xbsIndex_r4/Slice  nbits=21  boolean_output=off  mode=Upper Bit Location + Width  bit1=-294  base1=MSB of Input  bit0=0  base0=LSB of Input  dbl_ovrd=off  block_type=slice
  slice3 : xbsIndex_r4/Slice  nbits=21  boolean_output=off  mode=Upper Bit Location + Width  bit1=-273  base1=MSB of Input  bit0=0  base0=LSB of Input  dbl_ovrd=off  block_type=slice
  slice4 : xbsIndex_r4/Slice  nbits=21  boolean_output=off  mode=Upper Bit Location + Width  bit1=-252  base1=MSB of Input  bit0=0  base0=LSB of Input  dbl_ovrd=off  block_type=slice
  slice5 : xbsIndex_r4/Slice  nbits=21  boolean_output=off  mode=Upper Bit Location + Width  bit1=-231  base1=MSB of Input  bit0=0  base0=LSB of Input  dbl_ovrd=off  block_type=slice
  slice6 : xbsIndex_r4/Slice  nbits=21  boolean_output=off  mode=Upper Bit Location + Width  bit1=-210  base1=MSB of Input  bit0=0  base0=LSB of Input  dbl_ovrd=off  block_type=slice
  slice7 : xbsIndex_r4/Slice  nbits=21  boolean_output=off  mode=Upper Bit Location + Width  bit1=-189  base1=MSB of Input  bit0=0  base0=LSB of Input  dbl_ovrd=off  block_type=slice
  slice8 : xbsIndex_r4/Slice  nbits=21  boolean_output=off  mode=Upper Bit Location + Width  bit1=-168  base1=MSB of Input  bit0=0  base0=LSB of Input  dbl_ovrd=off  block_type=slice
  slice9 : xbsIndex_r4/Slice  nbits=21  boolean_output=off  mode=Upper Bit Location + Width  bit1=-147  base1=MSB of Input  bit0=0  base0=LSB of Input  dbl_ovrd=off  block_type=slice
  msb_out16 : Outport
  out15 : Outport  Port=2
  out14 : Outport  Port=3
  out13 : Outport  Port=4
  out12 : Outport  Port=5
  out11 : Outport  Port=6
  out10 : Outport  Port=7
  out9 : Outport  Port=8
  out8 : Outport  Port=9
  out7 : Outport  Port=10
  out6 : Outport  Port=11
  out5 : Outport  Port=12
  out4 : Outport  Port=13
  out3 : Outport  Port=14
  out2 : Outport  Port=15
  lsb_out1 : Outport  Port=16  VectorParamsAs1DForOutWhenUnconnected=off
  wires:
  reinterpret1/1 -> lsb_out1/1
  slice1/1 -> reinterpret1/1
  reinterpret2/1 -> out2/1
  slice2/1 -> reinterpret2/1
  reinterpret3/1 -> out3/1
  slice3/1 -> reinterpret3/1
  reinterpret4/1 -> out4/1
  slice4/1 -> reinterpret4/1
  reinterpret5/1 -> out5/1
  slice5/1 -> reinterpret5/1
  reinterpret6/1 -> out6/1
  slice6/1 -> reinterpret6/1
  reinterpret7/1 -> out7/1
  slice7/1 -> reinterpret7/1
  reinterpret8/1 -> out8/1
  slice8/1 -> reinterpret8/1
  reinterpret9/1 -> out9/1
  slice9/1 -> reinterpret9/1
  reinterpret10/1 -> out10/1
  slice10/1 -> reinterpret10/1
  reinterpret11/1 -> out11/1
  slice11/1 -> reinterpret11/1
  reinterpret12/1 -> out12/1
  slice12/1 -> reinterpret12/1
  reinterpret13/1 -> out13/1
  slice13/1 -> reinterpret13/1
  reinterpret14/1 -> out14/1
  slice14/1 -> reinterpret14/1
  reinterpret15/1 -> out15/1
  slice15/1 -> reinterpret15/1
  reinterpret16/1 -> msb_out16/1
  slice16/1 -> reinterpret16/1
  bus_in/1 -> slice1/1, slice2/1, slice3/1, slice4/1, slice5/1, slice6/1, slice7/1, slice8/1, slice9/1, slice10/1, slice11/1, slice12/1, slice13/1, slice14/1, slice15/1, slice16/1

== system rfsoc4x2_ospfb_128/fft_wideband_real1/fft_direct/butterfly1_1/bus_convert/of_bussify ==
  in1 : Inport
  in2 : Inport  Port=2
  in3 : Inport  Port=3
  in4 : Inport  Port=4
  in5 : Inport  Port=5
  in6 : Inport  Port=6
  in7 : Inport  Port=7
  in8 : Inport  Port=8
  in9 : Inport  Port=9
  in10 : Inport  Port=10
  in11 : Inport  Port=11
  in12 : Inport  Port=12
  in13 : Inport  Port=13
  in14 : Inport  Port=14
  in15 : Inport  Port=15
  in16 : Inport  Port=16
  concatenate : xbsIndex_r4/Concat  num_inputs=16  dbl_ovrd=off  block_type=concat
  reinterpret{1..16} (16 alike) : xbsIndex_r4/Reinterpret  force_arith_type=on  arith_type=Unsigned  force_bin_pt=on  bin_pt=0  block_type=reinterpret
      reinterpret1 settings: infoedit="Changes signal type without altering the binary representation.   You can changed the signal between signed and unsigned, and relocate the binary point.<br><br>Hardware notes: In hardware this block costs nothing.<br><br>Example:  Suppose the input is 6 bits wide, signed, with 2 fractional bits, and the output is forced to unsigned with 0 fractional bits.  Then an input of -2.0 (1110.00 in binary 2's complement) becomes an output of 56 (111000 in binary)."
      reinterpret2 settings: infoedit="Changes signal type without altering the binary representation.   You can changed the signal between signed and unsigned, and relocate the binary point.<br><br>Hardware notes: In hardware this block costs nothing.<br><br>Example:  Suppose the input is 6 bits wide, signed, with 2 fractional bits, and the output is forced to unsigned with 0 fractional bits.  Then an input of -2.0 (1110.00 in binary 2's complement) becomes an output of 56 (111000 in binary)."
  bus_out : Outport  VectorParamsAs1DForOutWhenUnconnected=off
  wires:
  reinterpret16/1 -> concatenate/16
  in16/1 -> reinterpret16/1
  reinterpret15/1 -> concatenate/15
  in15/1 -> reinterpret15/1
  reinterpret14/1 -> concatenate/14
  in14/1 -> reinterpret14/1
  reinterpret13/1 -> concatenate/13
  in13/1 -> reinterpret13/1
  reinterpret12/1 -> concatenate/12
  in12/1 -> reinterpret12/1
  reinterpret11/1 -> concatenate/11
  in11/1 -> reinterpret11/1
  reinterpret10/1 -> concatenate/10
  in10/1 -> reinterpret10/1
  reinterpret9/1 -> concatenate/9
  in9/1 -> reinterpret9/1
  reinterpret8/1 -> concatenate/8
  in8/1 -> reinterpret8/1
  reinterpret7/1 -> concatenate/7
  in7/1 -> reinterpret7/1
  reinterpret6/1 -> concatenate/6
  in6/1 -> reinterpret6/1
  reinterpret5/1 -> concatenate/5
  in5/1 -> reinterpret5/1
  reinterpret4/1 -> concatenate/4
  in4/1 -> reinterpret4/1
  reinterpret3/1 -> concatenate/3
  in3/1 -> reinterpret3/1
  reinterpret2/1 -> concatenate/2
  in2/1 -> reinterpret2/1
  reinterpret1/1 -> concatenate/1
  in1/1 -> reinterpret1/1
  concatenate/1 -> bus_out/1

== system rfsoc4x2_ospfb_128/fft_wideband_real1/fft_direct/butterfly1_1/bus_norm0/bussify ==
  in1 : Inport
  in2 : Inport  Port=2
  in3 : Inport  Port=3
  in4 : Inport  Port=4
  in5 : Inport  Port=5
  in6 : Inport  Port=6
  in7 : Inport  Port=7
  in8 : Inport  Port=8
  in9 : Inport  Port=9
  in10 : Inport  Port=10
  in11 : Inport  Port=11
  in12 : Inport  Port=12
  in13 : Inport  Port=13
  in14 : Inport  Port=14
  in15 : Inport  Port=15
  in16 : Inport  Port=16
  concatenate : xbsIndex_r4/Concat  num_inputs=16  dbl_ovrd=off  block_type=concat
  reinterpret{1..16} (16 alike) : xbsIndex_r4/Reinterpret  force_arith_type=on  arith_type=Unsigned  force_bin_pt=on  bin_pt=0  block_type=reinterpret
      reinterpret1 settings: infoedit="Changes signal type without altering the binary representation.   You can changed the signal between signed and unsigned, and relocate the binary point.<br><br>Hardware notes: In hardware this block costs nothing.<br><br>Example:  Suppose the input is 6 bits wide, signed, with 2 fractional bits, and the output is forced to unsigned with 0 fractional bits.  Then an input of -2.0 (1110.00 in binary 2's complement) becomes an output of 56 (111000 in binary)."
      reinterpret2 settings: infoedit="Changes signal type without altering the binary representation.   You can changed the signal between signed and unsigned, and relocate the binary point.<br><br>Hardware notes: In hardware this block costs nothing.<br><br>Example:  Suppose the input is 6 bits wide, signed, with 2 fractional bits, and the output is forced to unsigned with 0 fractional bits.  Then an input of -2.0 (1110.00 in binary 2's complement) becomes an output of 56 (111000 in binary)."
  bus_out : Outport  VectorParamsAs1DForOutWhenUnconnected=off
  wires:
  reinterpret16/1 -> concatenate/16
  in16/1 -> reinterpret16/1
  reinterpret15/1 -> concatenate/15
  in15/1 -> reinterpret15/1
  reinterpret14/1 -> concatenate/14
  in14/1 -> reinterpret14/1
  reinterpret13/1 -> concatenate/13
  in13/1 -> reinterpret13/1
  reinterpret12/1 -> concatenate/12
  in12/1 -> reinterpret12/1
  reinterpret11/1 -> concatenate/11
  in11/1 -> reinterpret11/1
  reinterpret10/1 -> concatenate/10
  in10/1 -> reinterpret10/1
  reinterpret9/1 -> concatenate/9
  in9/1 -> reinterpret9/1
  reinterpret8/1 -> concatenate/8
  in8/1 -> reinterpret8/1
  reinterpret7/1 -> concatenate/7
  in7/1 -> reinterpret7/1
  reinterpret6/1 -> concatenate/6
  in6/1 -> reinterpret6/1
  reinterpret5/1 -> concatenate/5
  in5/1 -> reinterpret5/1
  reinterpret4/1 -> concatenate/4
  in4/1 -> reinterpret4/1
  reinterpret3/1 -> concatenate/3
  in3/1 -> reinterpret3/1
  reinterpret2/1 -> concatenate/2
  in2/1 -> reinterpret2/1
  reinterpret1/1 -> concatenate/1
  in1/1 -> reinterpret1/1
  concatenate/1 -> bus_out/1

== system rfsoc4x2_ospfb_128/fft_wideband_real1/fft_direct/butterfly1_1/bus_norm0/debus ==
  bus_in : Inport
  reinterpret{1..16} (16 alike) : xbsIndex_r4/Reinterpret  force_arith_type=on  arith_type="Signed  (2's comp)"  force_bin_pt=on  bin_pt=17  block_type=reinterpret
  slice1 : xbsIndex_r4/Slice  nbits=20  boolean_output=off  mode=Upper Bit Location + Width  bit1=-300  base1=MSB of Input  bit0=0  base0=LSB of Input  dbl_ovrd=off  block_type=slice
  slice10 : xbsIndex_r4/Slice  nbits=20  boolean_output=off  mode=Upper Bit Location + Width  bit1=-120  base1=MSB of Input  bit0=0  base0=LSB of Input  dbl_ovrd=off  block_type=slice
  slice11 : xbsIndex_r4/Slice  nbits=20  boolean_output=off  mode=Upper Bit Location + Width  bit1=-100  base1=MSB of Input  bit0=0  base0=LSB of Input  dbl_ovrd=off  block_type=slice
  slice12 : xbsIndex_r4/Slice  nbits=20  boolean_output=off  mode=Upper Bit Location + Width  bit1=-80  base1=MSB of Input  bit0=0  base0=LSB of Input  dbl_ovrd=off  block_type=slice
  slice13 : xbsIndex_r4/Slice  nbits=20  boolean_output=off  mode=Upper Bit Location + Width  bit1=-60  base1=MSB of Input  bit0=0  base0=LSB of Input  dbl_ovrd=off  block_type=slice
  slice14 : xbsIndex_r4/Slice  nbits=20  boolean_output=off  mode=Upper Bit Location + Width  bit1=-40  base1=MSB of Input  bit0=0  base0=LSB of Input  dbl_ovrd=off  block_type=slice
  slice15 : xbsIndex_r4/Slice  nbits=20  boolean_output=off  mode=Upper Bit Location + Width  bit1=-20  base1=MSB of Input  bit0=0  base0=LSB of Input  dbl_ovrd=off  block_type=slice
  slice16 : xbsIndex_r4/Slice  nbits=20  boolean_output=off  mode=Upper Bit Location + Width  bit1=0  base1=MSB of Input  bit0=0  base0=LSB of Input  dbl_ovrd=off  block_type=slice
  slice2 : xbsIndex_r4/Slice  nbits=20  boolean_output=off  mode=Upper Bit Location + Width  bit1=-280  base1=MSB of Input  bit0=0  base0=LSB of Input  dbl_ovrd=off  block_type=slice
  slice3 : xbsIndex_r4/Slice  nbits=20  boolean_output=off  mode=Upper Bit Location + Width  bit1=-260  base1=MSB of Input  bit0=0  base0=LSB of Input  dbl_ovrd=off  block_type=slice
  slice4 : xbsIndex_r4/Slice  nbits=20  boolean_output=off  mode=Upper Bit Location + Width  bit1=-240  base1=MSB of Input  bit0=0  base0=LSB of Input  dbl_ovrd=off  block_type=slice
  slice5 : xbsIndex_r4/Slice  nbits=20  boolean_output=off  mode=Upper Bit Location + Width  bit1=-220  base1=MSB of Input  bit0=0  base0=LSB of Input  dbl_ovrd=off  block_type=slice
  slice6 : xbsIndex_r4/Slice  nbits=20  boolean_output=off  mode=Upper Bit Location + Width  bit1=-200  base1=MSB of Input  bit0=0  base0=LSB of Input  dbl_ovrd=off  block_type=slice
  slice7 : xbsIndex_r4/Slice  nbits=20  boolean_output=off  mode=Upper Bit Location + Width  bit1=-180  base1=MSB of Input  bit0=0  base0=LSB of Input  dbl_ovrd=off  block_type=slice
  slice8 : xbsIndex_r4/Slice  nbits=20  boolean_output=off  mode=Upper Bit Location + Width  bit1=-160  base1=MSB of Input  bit0=0  base0=LSB of Input  dbl_ovrd=off  block_type=slice
  slice9 : xbsIndex_r4/Slice  nbits=20  boolean_output=off  mode=Upper Bit Location + Width  bit1=-140  base1=MSB of Input  bit0=0  base0=LSB of Input  dbl_ovrd=off  block_type=slice
  msb_out16 : Outport
  out15 : Outport  Port=2
  out14 : Outport  Port=3
  out13 : Outport  Port=4
  out12 : Outport  Port=5
  out11 : Outport  Port=6
  out10 : Outport  Port=7
  out9 : Outport  Port=8
  out8 : Outport  Port=9
  out7 : Outport  Port=10
  out6 : Outport  Port=11
  out5 : Outport  Port=12
  out4 : Outport  Port=13
  out3 : Outport  Port=14
  out2 : Outport  Port=15
  lsb_out1 : Outport  Port=16  VectorParamsAs1DForOutWhenUnconnected=off
  wires:
  reinterpret1/1 -> lsb_out1/1
  slice1/1 -> reinterpret1/1
  reinterpret2/1 -> out2/1
  slice2/1 -> reinterpret2/1
  reinterpret3/1 -> out3/1
  slice3/1 -> reinterpret3/1
  reinterpret4/1 -> out4/1
  slice4/1 -> reinterpret4/1
  reinterpret5/1 -> out5/1
  slice5/1 -> reinterpret5/1
  reinterpret6/1 -> out6/1
  slice6/1 -> reinterpret6/1
  reinterpret7/1 -> out7/1
  slice7/1 -> reinterpret7/1
  reinterpret8/1 -> out8/1
  slice8/1 -> reinterpret8/1
  reinterpret9/1 -> out9/1
  slice9/1 -> reinterpret9/1
  reinterpret10/1 -> out10/1
  slice10/1 -> reinterpret10/1
  reinterpret11/1 -> out11/1
  slice11/1 -> reinterpret11/1
  reinterpret12/1 -> out12/1
  slice12/1 -> reinterpret12/1
  reinterpret13/1 -> out13/1
  slice13/1 -> reinterpret13/1
  reinterpret14/1 -> out14/1
  slice14/1 -> reinterpret14/1
  reinterpret15/1 -> out15/1
  slice15/1 -> reinterpret15/1
  reinterpret16/1 -> msb_out16/1
  slice16/1 -> reinterpret16/1
  bus_in/1 -> slice1/1, slice2/1, slice3/1, slice4/1, slice5/1, slice6/1, slice7/1, slice8/1, slice9/1, slice10/1, slice11/1, slice12/1, slice13/1, slice14/1, slice15/1, slice16/1

== system rfsoc4x2_ospfb_128/fft_wideband_real1/fft_direct/butterfly1_1/bus_norm1/bussify ==
  in1 : Inport
  in2 : Inport  Port=2
  in3 : Inport  Port=3
  in4 : Inport  Port=4
  in5 : Inport  Port=5
  in6 : Inport  Port=6
  in7 : Inport  Port=7
  in8 : Inport  Port=8
  in9 : Inport  Port=9
  in10 : Inport  Port=10
  in11 : Inport  Port=11
  in12 : Inport  Port=12
  in13 : Inport  Port=13
  in14 : Inport  Port=14
  in15 : Inport  Port=15
  in16 : Inport  Port=16
  concatenate : xbsIndex_r4/Concat  num_inputs=16  dbl_ovrd=off  block_type=concat
  reinterpret{1..16} (16 alike) : xbsIndex_r4/Reinterpret  force_arith_type=on  arith_type=Unsigned  force_bin_pt=on  bin_pt=0  block_type=reinterpret
      reinterpret1 settings: infoedit="Changes signal type without altering the binary representation.   You can changed the signal between signed and unsigned, and relocate the binary point.<br><br>Hardware notes: In hardware this block costs nothing.<br><br>Example:  Suppose the input is 6 bits wide, signed, with 2 fractional bits, and the output is forced to unsigned with 0 fractional bits.  Then an input of -2.0 (1110.00 in binary 2's complement) becomes an output of 56 (111000 in binary)."
      reinterpret2 settings: infoedit="Changes signal type without altering the binary representation.   You can changed the signal between signed and unsigned, and relocate the binary point.<br><br>Hardware notes: In hardware this block costs nothing.<br><br>Example:  Suppose the input is 6 bits wide, signed, with 2 fractional bits, and the output is forced to unsigned with 0 fractional bits.  Then an input of -2.0 (1110.00 in binary 2's complement) becomes an output of 56 (111000 in binary)."
  bus_out : Outport  VectorParamsAs1DForOutWhenUnconnected=off
  wires:
  reinterpret16/1 -> concatenate/16
  in16/1 -> reinterpret16/1
  reinterpret15/1 -> concatenate/15
  in15/1 -> reinterpret15/1
  reinterpret14/1 -> concatenate/14
  in14/1 -> reinterpret14/1
  reinterpret13/1 -> concatenate/13
  in13/1 -> reinterpret13/1
  reinterpret12/1 -> concatenate/12
  in12/1 -> reinterpret12/1
  reinterpret11/1 -> concatenate/11
  in11/1 -> reinterpret11/1
  reinterpret10/1 -> concatenate/10
  in10/1 -> reinterpret10/1
  reinterpret9/1 -> concatenate/9
  in9/1 -> reinterpret9/1
  reinterpret8/1 -> concatenate/8
  in8/1 -> reinterpret8/1
  reinterpret7/1 -> concatenate/7
  in7/1 -> reinterpret7/1
  reinterpret6/1 -> concatenate/6
  in6/1 -> reinterpret6/1
  reinterpret5/1 -> concatenate/5
  in5/1 -> reinterpret5/1
  reinterpret4/1 -> concatenate/4
  in4/1 -> reinterpret4/1
  reinterpret3/1 -> concatenate/3
  in3/1 -> reinterpret3/1
  reinterpret2/1 -> concatenate/2
  in2/1 -> reinterpret2/1
  reinterpret1/1 -> concatenate/1
  in1/1 -> reinterpret1/1
  concatenate/1 -> bus_out/1
